simulink model "TVCmodel"  (R2025b)
settings: Solver=VariableStepAuto  StartTime=0.0  StopTime=20  RelTol=1e-3
values from neighbouring files (symbols this model uses):
  initialCondition = [0,0,0,0,0,0,0,0,0,0,0,0]    [Simulate.m]
  Ka = lqr(A,B,Q,R)    [FindAttitudeGainMatrix.m]    (also in Simulate.m = FindAttitudeGainMatrix([0,0,0,0,0,0],[0,0,0],constants,9.81,)
  Kp = lqr(A,B,Q,R)    [FindPositionGainMatrix.m]    (also in Simulate.m = FindPositionGainMatrix([0,0,0,0,0,0],[0,0,0],constants,Qp,Rp)
  posTgt = [1,0,-50,0,0,0]    [Simulate.m]
settings Model: Creator=lucas  LastModifiedBy=lucas

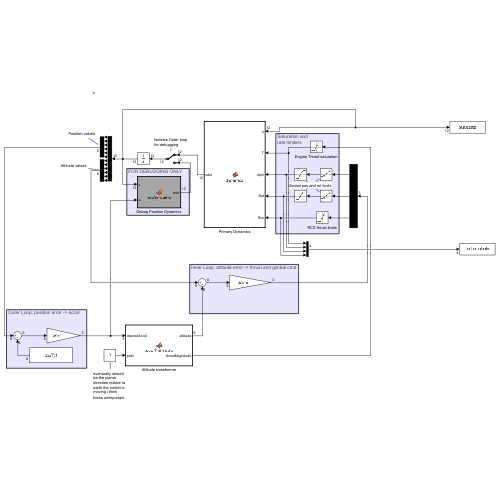
[thumbnail: Simulink's stored preview of the top-level diagram]
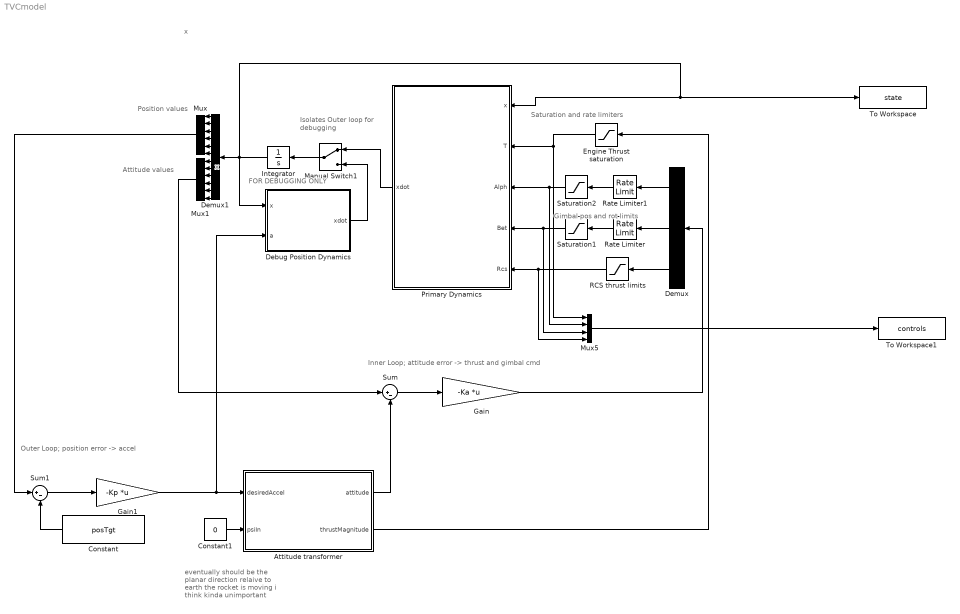
== system TVCmodel ==
  note: Gimbal pos and rot limits
  note: Attitude values
  note: Saturation and
      | rate limiters
  note: eventually should be the planar direction relaive to earth the rocket is moving i think
      | kinda unimportant
  note: FOR DEBUGGING ONLY
  note: Isolates Outer loop
      | for debugging
  note: Outer Loop; position error -> accel
  note: Inner Loop; attitude error -> thrust and gimbal cmd
  note: x
  note: x
  note: Position values
  Attitude transformer : MATLAB Function  TreatAsAtomicUnit=on
  Constant : Constant  Value=posTgt
  Constant1 : Constant  Value=0
  Debug Position Dynamics : MATLAB Function  TreatAsAtomicUnit=on
  Demux : Demux  Outputs=3
  Demux1 : Demux  Outputs=12
  Engine Thrust saturation : Saturate  UpperLimit=2891  LowerLimit=0
  Gain : Gain  Gain=-Ka  Multiplication=Matrix(K*u)
  Gain1 : Gain  Gain=-Kp  Multiplication=Matrix(K*u)
  Integrator : Integrator  InitialCondition=initialCondition
  Manual Switch1 : ManualSwitch
  Mux : Mux  Inputs=6
  Mux1 : Mux  Inputs=6
  Mux5 : Mux
  Primary Dynamics : MATLAB Function  TreatAsAtomicUnit=on
  RCS thrust limits : Saturate
  Rate Limiter : RateLimiter  RisingSlewLimit=8  FallingSlewLimit=-8  SampleTimeMode=inherited
  Rate Limiter1 : RateLimiter  RisingSlewLimit=8  FallingSlewLimit=-8  SampleTimeMode=inherited
  Saturation1 : Saturate  UpperLimit=0.17  LowerLimit=-0.17
  Saturation2 : Saturate  UpperLimit=0.17  LowerLimit=-0.17
  Sum : Sum  Inputs=|+-
  Sum1 : Sum  Inputs=|+-
  To Workspace : ToWorkspace  VariableName=state  SampleTime=-1
  To Workspace1 : ToWorkspace  VariableName=controls  SampleTime=-1
  wires:
  Demux1/1 -> Mux/1
  Demux1/2 -> Mux/2
  Demux1/4 -> Mux/4
  Demux1/3 -> Mux/3
  Demux1/5 -> Mux/5
  Demux1/6 -> Mux/6
  Demux1/7 -> Mux1/1
  Demux1/8 -> Mux1/2
  Demux1/9 -> Mux1/3
  Demux1/10 -> Mux1/4
  Demux1/11 -> Mux1/5
  Demux1/12 -> Mux1/6
  Integrator/1 -> Debug Position Dynamics/1(x), To Workspace/1, Primary Dynamics/1(x), Demux1/1
  Sum/1 -> Gain/1
  Mux1/1 -> Sum/1
  Gain/1 -> Demux/1
  Gain1/1 -> Debug Position Dynamics/2(a), Attitude transformer/1(desiredAccel)
  Sum1/1 -> Gain1/1
  Manual Switch1/1 -> Integrator/1
  Primary Dynamics/1(xdot) -> Manual Switch1/1
  Attitude transformer/2(thrustMagnitude) -> Engine Thrust saturation/1
  Attitude transformer/1(attitude) -> Sum/2
  Debug Position Dynamics/1(xdot) -> Manual Switch1/2
  Demux/1 -> Rate Limiter1/1
  Demux/2 -> Rate Limiter/1
  Demux/3 -> RCS thrust limits/1
  Engine Thrust saturation/1 -> Primary Dynamics/2(T), Mux5/1
  Saturation1/1 -> Mux5/3, Primary Dynamics/4(Bet)
  Saturation2/1 -> Mux5/2, Primary Dynamics/3(Alph)
  Rate Limiter/1 -> Saturation1/1
  Rate Limiter1/1 -> Saturation2/1
  Mux/1 -> Sum1/1
  Constant/1 -> Sum1/2
  Mux5/1 -> To Workspace1/1
  Constant1/1 -> Attitude transformer/2(psiIn)
  RCS thrust limits/1 -> Mux5/4, Primary Dynamics/5(Rcs)

== matlab function TVCmodel/Attitude transformer ==
  data: desiredAccel input size=[3,1]; attitude output size=6; thrustMagnitude output; constants parameter; psiIn input
function [attitude,thrustMagnitude] = AccelToAttitude(desiredAccel, constants, psiIn)
arguments
    desiredAccel (3,1) double
    constants (6,1) double
    psiIn (1,1) double
end

    %Function that takes in desired acceleration and outputs what thrust 
    % and direction the rocket should point in to achieve that, and cancel 
    % gravity.
    

    %so i think this code needs to be changed if we want to add other
    %disturbance forces aside from gravity? im not sure though. mabye not
    %because this is just supposed to be a baseline, it should be able to
    %compensate from the error.


    %quick aliases
    m=constants(1); g=constants(2);

    

    %find the force required to both counter gravity and accelerate in
    %desired direction
    desiredThrust = m*g*[0;0;1] - m*desiredAccel;

    thrustMagnitude = norm(desiredThrust);

    %to prevent div/0
    if thrustMagnitude < 1e-9
        desiredThrust = g*[0;0;1];
        thrustMagnitude = norm(desiredThrust);
    end
    
    

    %unit vector pointing from back of rocket
    desiredThrustDir = desiredThrust/thrustMagnitude;
    
    %basically zero forever right now, supposedly having psiCmd go towards
    %where the rocket is pointing is a better implementation
    yawHeading = [cos(psiIn); sin(psiIn); 0];

    % math for making a rotation matrix that goes from world frame to a
    % frame with pos z towards the rear of the rocket, and with positive X
    % in the direction of psi
    c = cross(desiredThrustDir,yawHeading);

    if norm(c)<1e-6
        yawHeading = [cos(psiIn+0.1); sin(psiIn+0.1); 0];
        c = cross(desiredThrustDir,yawHeading);
    end
    %create frame pointing in desired thrust direction
    frameDir2 = c/norm(c);
    frameDir1 = cross(frameDir2,desiredThrustDir);
    frame = [frameDir1 frameDir2 desiredThrustDir];
    
    %turn that frame into desired euler angles
    thetaCmd = asin(-frame(3,1));
    phiCmd   = atan2(frame(3,2), frame(3,3));
    psiCmd   = psiIn;
    % no psi command rn, technically would be best if it took the direction
    % the rocket was traveling but thats for a later date. instead just
    % pass through

    %output as column vector for simulink and convention, zeros are just to
    %make it fit the state vector in the sum block
    attitude = [phiCmd;thetaCmd;psiCmd;0;0;0];
end

== matlab function TVCmodel/Primary Dynamics ==
  data: x input; xdot output size=12; T input; Alph input; Bet input; Rcs input; constants parameter
function xdot = dynamics(x, T, Alph, Bet, Rcs, constants)
%full dynamics for attitude and position

%not well comented but its pretty self explanatory ngl

%output as column vector for simulink and convention
xdot = [0;0;0;0;0;0;0;0;0;0;0;0];

% ew, just ew, but its cleaner than assigning each individually, idk if its
% more optimized though
[cell] = num2cell(constants);
[m g L Ixx Iyy Izz] = deal(cell{:});

pn = x(1);
pe = x(2);
pd = x(3);
u = x(4);
v = x(5);
w = x(6);
Phi = x(7);
Theta = x(8);
Psi = x(9);
p = x(10);
q = x(11);
r = x(12);

%p_n
xdot(1) = cos(Theta)*cos(Psi)*u + (sin(Phi)*sin(Theta)*cos(Psi) - cos(Phi)*sin(Psi))*v + (cos(Phi)*sin(Theta)*cos(Psi) + sin(Phi)*sin(Psi))*w;
%p_e
xdot(2) = cos(Theta)*sin(Psi)*u + (sin(Phi)*sin(Theta)*sin(Psi) + cos(Phi)*cos(Psi))*v + (cos(Phi)*sin(Theta)*sin(Psi) - sin(Phi)*cos(Psi))*w;
%h
xdot(3) = -(sin(Theta)*u - sin(Phi)*cos(Theta)*v - cos(Phi)*cos(Theta)*w);
%u
xdot(4) = r*v - q*w + (T*sin(Bet)*cos(Alph) - m*g*sin(Theta))/m;
%v
xdot(5) = p*w - r*u + (-T*sin(Alph)*cos(Bet) + m*g*cos(Theta)*sin(Phi))/m;
%w
xdot(6) = q*u - p*v + (-T*cos(Alph)*cos(Bet) + m*g*cos(Theta)*cos(Phi))/m;
%phi 
xdot(7) = p + sin(Phi)*tan(Theta)*q + cos(Phi)*tan(Theta)*r;
%theta
xdot(8) = cos(Phi)*q - sin(Phi)*r;
%psi
xdot(9) =  (sin(Phi)/cos(Theta))*q + (cos(Phi)/cos(Theta))*r;
%p
xdot(10) = (Iyy - Izz)*q*r/Ixx + (L*T*sin(Alph)*cos(Bet))/Ixx;
%q
xdot(11) = (Izz - Ixx)*p*r/Iyy - (L*T*sin(Bet)*cos(Alph))/Iyy;
%r
xdot(12) = (Ixx - Iyy)*p*q/Izz + Rcs/Izz;
end

== matlab function TVCmodel/Debug Position Dynamics ==
  data: x input; xdot output size=12; a input
function xdot = posDynamics(x, a)
%simple dynamics for testing outer loop

%honestly so simple not gonna comment it

ax=a(1)
ay=a(2)
az=a(3)

%output as column vector for simulink and convention
xdot = [0;0;0;0;0;0;0;0;0;0;0;0];

pn = x(1);
pe = x(2);
h = x(3);
u = x(4);
v = x(5);
w = x(6);
Phi = x(7);
Theta = x(8);
Psi = x(9);
p = x(10);
q = x(11);
r = x(12);

%p_n
xdot(1) = u;
%p_e
xdot(2) = v;
%h
xdot(3) = w;
%u
xdot(4) = ax;
%v
xdot(5) = ay;
%w
xdot(6) = az;
end
